simulink model "physical_lab6_lead_example2"  (R2024b)
settings: Solver=ode15s  StartTime=0.0  StopTime=5  MaxStep=0.0016666666666666668  RelTol=1e-7  AbsTol=1e-9
model workspace (MAT data in the model file):
  physical_input = timeseries
  physical_input.Name = 'unnamed'
  physical_input.DataInfo = tsdata.datametadata
  physical_input.DataInfo.Interpolation = tsdata.interpolation
  physical_input.DataInfo.Interpolation.Fhandle : function handle (value not decoded)
  physical_input.DataInfo.Interpolation.Name = 'linear'
  physical_input.TimeInfo = tsdata.timemetadata
  physical_input.TimeInfo.Length = 3001
  physical_input.TimeInfo.DuplicateTimes = 0
  physical_input.TimeInfo.Time_ = [0 0.00166666666667 0.00333333333333 0.005 0.00666666666667 0.00833333333333 0.01 0.0116666666667 0.0133333333333 0.015 0.0166666666667 0.0183333333333 ... (3001 elements, 3001x1)]
  physical_input.TimeInfo.Initialized = 1
  physical_input.QualityInfo = tsdata.qualmetadata
  physical_input.Data_ = [0 0.0833333333333 0.166666666667 0.25 0.333333333333 0.416666666667 0.5 0.583333333333 0.666666666667 0.75 0.833333333333 0.916666666667 ... (3001 elements, 3001x1)]
libraries: fl_lib x38, nesl_utility x5
settings Model: Creator=33657  LastModifiedBy=33657

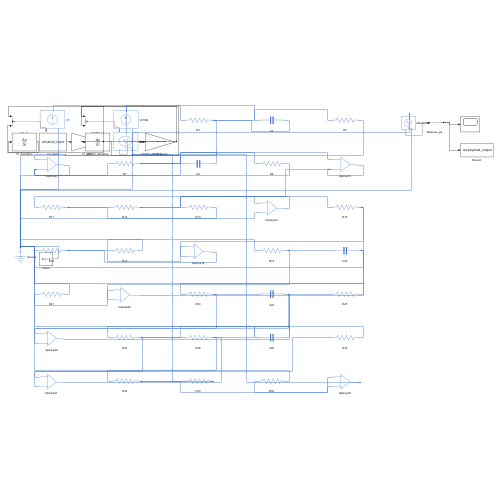
[thumbnail: Simulink's stored preview of the top-level diagram]
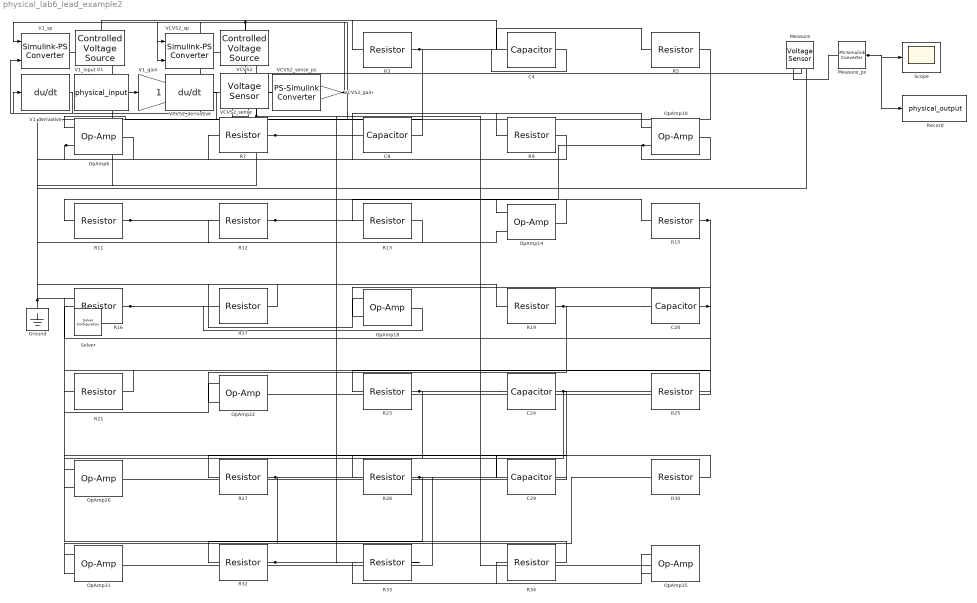
== system physical_lab6_lead_example2 ==
  C20 : fl_lib/Electrical/Electrical Elements/Capacitor  c=1.0000000000000001e-05 F  r=0 Ohm  g=0 1/Ohm  i_specify=off  i_priority=None  i=0 A  i_nominal_specify=off  i_nominal_value=1  i_nominal_unit=A  v_specify=off  v_priority=None  v=0 V  v_nominal_specify=off  v_nominal_value=1  v_nominal_unit=V  vc_specify=off  vc_priority=High  vc=0 V  vc_nominal_specify=off  vc_nominal_value=1  vc_nominal_unit=V
  C24 : fl_lib/Electrical/Electrical Elements/Capacitor  c=1.0000000000000001e-05 F  r=0 Ohm  g=0 1/Ohm  i_specify=off  i_priority=None  i=0 A  i_nominal_specify=off  i_nominal_value=1  i_nominal_unit=A  v_specify=off  v_priority=None  v=0 V  v_nominal_specify=off  v_nominal_value=1  v_nominal_unit=V  vc_specify=off  vc_priority=High  vc=0 V  vc_nominal_specify=off  vc_nominal_value=1  vc_nominal_unit=V
  C29 : fl_lib/Electrical/Electrical Elements/Capacitor  c=1.9999999999999999e-06 F  r=0 Ohm  g=0 1/Ohm  i_specify=off  i_priority=None  i=0 A  i_nominal_specify=off  i_nominal_value=1  i_nominal_unit=A  v_specify=off  v_priority=None  v=0 V  v_nominal_specify=off  v_nominal_value=1  v_nominal_unit=V  vc_specify=off  vc_priority=High  vc=0 V  vc_nominal_specify=off  vc_nominal_value=1  vc_nominal_unit=V
  C4 : fl_lib/Electrical/Electrical Elements/Capacitor  c=9.9999999999999995e-07 F  r=0 Ohm  g=0 1/Ohm  i_specify=off  i_priority=None  i=0 A  i_nominal_specify=off  i_nominal_value=1  i_nominal_unit=A  v_specify=off  v_priority=None  v=0 V  v_nominal_specify=off  v_nominal_value=1  v_nominal_unit=V  vc_specify=off  vc_priority=High  vc=0 V  vc_nominal_specify=off  vc_nominal_value=1  vc_nominal_unit=V
  C8 : fl_lib/Electrical/Electrical Elements/Capacitor  c=9.9999999999999995e-07 F  r=0 Ohm  g=0 1/Ohm  i_specify=off  i_priority=None  i=0 A  i_nominal_specify=off  i_nominal_value=1  i_nominal_unit=A  v_specify=off  v_priority=None  v=0 V  v_nominal_specify=off  v_nominal_value=1  v_nominal_unit=V  vc_specify=off  vc_priority=High  vc=0 V  vc_nominal_specify=off  vc_nominal_value=1  vc_nominal_unit=V
  Ground : fl_lib/Electrical/Electrical Elements/Electrical Reference
  Measure : fl_lib/Electrical/Electrical Sensors/Voltage Sensor
  Measure_ps : nesl_utility/PS-Simulink Converter  PhysicalDomain=network_engine_domain  SubClassName=ps_output  LeftPortType=input  RightPortType=output  PseudoPeriodic=off  Frequencies=[]  VectorFormat=inherit  Unit=V  AffineConversion=off
  OpAmp{6,10,14,18,22,26,31,35} (8 alike) : fl_lib/Electrical/Electrical Elements/Op-Amp  outI_specify=off  outI_priority=None  outI=0 A  outI_nominal_specify=off  outI_nominal_value=1  outI_nominal_unit=A
  R{11,13,15..17,19,21,23,25,27..28,30,32,34} (14 alike) : fl_lib/Electrical/Electrical Elements/Resistor  R=100000 Ohm  i_specify=off  i_priority=None  i=0 A  i_nominal_specify=off  i_nominal_value=1  i_nominal_unit=A  v_specify=off  v_priority=None  v=0 V  v_nominal_specify=off  v_nominal_value=1  v_nominal_unit=V
  R12 : fl_lib/Electrical/Electrical Elements/Resistor  R=3600000 Ohm  i_specify=off  i_priority=None  i=0 A  i_nominal_specify=off  i_nominal_value=1  i_nominal_unit=A  v_specify=off  v_priority=None  v=0 V  v_nominal_specify=off  v_nominal_value=1  v_nominal_unit=V
  R3 : fl_lib/Electrical/Electrical Elements/Resistor  R=408248.290463863 Ohm  i_specify=off  i_priority=None  i=0 A  i_nominal_specify=off  i_nominal_value=1  i_nominal_unit=A  v_specify=off  v_priority=None  v=0 V  v_nominal_specify=off  v_nominal_value=1  v_nominal_unit=V
  R33 : fl_lib/Electrical/Electrical Elements/Resistor  R=1000000 Ohm  i_specify=off  i_priority=None  i=0 A  i_nominal_specify=off  i_nominal_value=1  i_nominal_unit=A  v_specify=off  v_priority=None  v=0 V  v_nominal_specify=off  v_nominal_value=1  v_nominal_unit=V
  R5 : fl_lib/Electrical/Electrical Elements/Resistor  R=81649.658092772603 Ohm  i_specify=off  i_priority=None  i=0 A  i_nominal_specify=off  i_nominal_value=1  i_nominal_unit=A  v_specify=off  v_priority=None  v=0 V  v_nominal_specify=off  v_nominal_value=1  v_nominal_unit=V
  R7 : fl_lib/Electrical/Electrical Elements/Resistor  R=408248.290463863 Ohm  i_specify=off  i_priority=None  i=0 A  i_nominal_specify=off  i_nominal_value=1  i_nominal_unit=A  v_specify=off  v_priority=None  v=0 V  v_nominal_specify=off  v_nominal_value=1  v_nominal_unit=V
  R9 : fl_lib/Electrical/Electrical Elements/Resistor  R=81649.658092772603 Ohm  i_specify=off  i_priority=None  i=0 A  i_nominal_specify=off  i_nominal_value=1  i_nominal_unit=A  v_specify=off  v_priority=None  v=0 V  v_nominal_specify=off  v_nominal_value=1  v_nominal_unit=V
  Record : ToWorkspace  VariableName=physical_output  SaveFormat=Timeseries  SampleTime=-1
  Scope : Scope
  Solver : nesl_utility/Solver Configuration  PhysicalDomain=network_engine_domain  SubClassName=solver  LeftPortType=input  RightPortType=generic  Tones=[]  Harmonics=[]  SimulateNoise=off  Profile=off  UseLocalSampling=off  EnableSwitchedLinearOptims=on  FrequencyDomain=off  UseCCode=off  RelTol=0.001  AbsTol=0.001  MinStep=1e-09  ToWorkspace=off  RevertToSquareIcSolve=off  NumHomotopyIterations=100  PhasorMode=off  PhasorModeNumHarmonics=1  ConsistencySolver=NEWTON_XTOL_AFTER_FTOL  IndexReductionMethod=DerivativeReplacement  DoDC=off  ResidualTolerance=1e-09  ConsistencyTolSource=GLOBAL  ConsistencyAbsTol=0.001  ConsistencyRelTol=0.001  ConsistencyTolFactor=0.001  UseLocalSolver=off  LocalSolverChoice=NE_BACKWARD_EULER_ADVANCER  ResolveIndetEquations=on  FunctionEvalNumThread=1  LocalSolverSampleTime=0.001  DoFixedCost=off  MaxNonlinIter=3  MaxModeIter=2  ComputeImpulses=off  ImpulseIterations=2  LinearAlgebra=auto  LinearAlgebraNumThread=0  EquationFormulation=NE_TIME_EF  DelaysMemoryBudget=1024  AutomaticFiltering=on  FilteringTimeConstant=0.001  PartitionStorageMethod=AS_NEEDED  PartitionMemoryBudget=1024  PartitionMethod=ROBUST  MultibodyUseLocalSolver=off  MultibodyLocalSolverChoice=ODE1  MultibodyLocalSolverSampleTime=0.001
  V1 : fl_lib/Electrical/Electrical Sources/Controlled Voltage Source
  V1_derivative : Derivative
  V1_gain : Gain
  V1_input : FromWorkspace  VariableName=physical_input
  V1_sp : nesl_utility/Simulink-PS Converter  PhysicalDomain=network_engine_domain  SubClassName=ps_input  LeftPortType=input  RightPortType=output  PseudoPeriodic=off  Frequencies=[]  NoiseDistribution=none  NoiseParameters=[]  Unit=V  AffineConversion=off  FilteringAndDerivatives=provide  SimscapeFilterOrder=1  InputFilterTimeConstant=0.001  UdotUserProvided=1
  VCVS2 : fl_lib/Electrical/Electrical Sources/Controlled Voltage Source
  VCVS2_derivative : Derivative
  VCVS2_gain : Gain
  VCVS2_sense : fl_lib/Electrical/Electrical Sensors/Voltage Sensor
  VCVS2_sense_ps : nesl_utility/PS-Simulink Converter  PhysicalDomain=network_engine_domain  SubClassName=ps_output  LeftPortType=input  RightPortType=output  PseudoPeriodic=off  Frequencies=[]  VectorFormat=inherit  Unit=V  AffineConversion=off
  VCVS2_sp : nesl_utility/Simulink-PS Converter  PhysicalDomain=network_engine_domain  SubClassName=ps_input  LeftPortType=input  RightPortType=output  PseudoPeriodic=off  Frequencies=[]  NoiseDistribution=none  NoiseParameters=[]  Unit=V  AffineConversion=off  FilteringAndDerivatives=provide  SimscapeFilterOrder=1  InputFilterTimeConstant=0.001  UdotUserProvided=1
  wires:
  V1_input/1 -> V1_gain/1
  V1_gain/1 -> V1_derivative/1, V1_sp/1
  V1_derivative/1 -> V1_sp/2
  VCVS2_sense_ps/1 -> VCVS2_gain/1
  VCVS2_gain/1 -> VCVS2_derivative/1, VCVS2_sp/1
  VCVS2_derivative/1 -> VCVS2_sp/2
  Measure_ps/1 -> Scope/1, Record/1
  connections:
  Solver/RConn1 -- Ground/LConn1 -- V1/RConn2 -- VCVS2/RConn2 -- R5/RConn1 -- R9/RConn1 -- R13/RConn1 -- R17/RConn1 -- R21/RConn1 -- R25/RConn1 -- R30/RConn1 -- R34/RConn1 -- Measure/RConn2
  V1_sp/RConn1 -- V1/RConn1
  V1/LConn1 -- VCVS2_sense/LConn1
  VCVS2_sense/RConn1 -- VCVS2_sense_ps/LConn1
  VCVS2_sp/RConn1 -- VCVS2/RConn1
  R3/LConn1 -- VCVS2/LConn1 -- C4/LConn1
  C4/RConn1 -- R3/RConn1 -- R5/LConn1 -- OpAmp6/LConn1
  OpAmp6/RConn1 -- OpAmp6/LConn2 -- R7/LConn1 -- C8/LConn1
  C8/RConn1 -- R7/RConn1 -- R9/LConn1 -- OpAmp10/LConn1
  OpAmp10/RConn1 -- OpAmp10/LConn2 -- R11/LConn1
  R12/LConn1 -- R11/RConn1 -- OpAmp14/LConn2
  R13/LConn1 -- OpAmp14/LConn1
  OpAmp14/RConn1 -- R12/RConn1 -- R15/LConn1
  R16/LConn1 -- R15/RConn1 -- OpAmp18/LConn2
  R17/LConn1 -- OpAmp18/LConn1
  OpAmp18/RConn1 -- R16/RConn1 -- R19/LConn1
  C20/LConn1 -- R19/RConn1 -- OpAmp22/LConn2
  R21/LConn1 -- OpAmp22/LConn1
  OpAmp22/RConn1 -- C20/RConn1 -- R23/LConn1
  C24/LConn1 -- R23/RConn1 -- OpAmp26/LConn2
  R25/LConn1 -- OpAmp26/LConn1
  OpAmp26/RConn1 -- C24/RConn1 -- R27/LConn1
  R28/LConn1 -- R27/RConn1 -- C29/LConn1 -- OpAmp31/LConn2
  C29/RConn1 -- R28/RConn1 -- OpAmp31/RConn1 -- R32/LConn1
  R30/LConn1 -- OpAmp31/LConn1
  R33/LConn1 -- R32/RConn1 -- OpAmp35/LConn2
  R33/RConn1 -- VCVS2_sense/RConn2 -- OpAmp35/RConn1 -- Measure/LConn1
  R34/LConn1 -- OpAmp35/LConn1
  Measure/RConn1 -- Measure_ps/LConn1
